simulink model "tdpSingleRobot"  (R2026b)
settings: Solver=FixedStepDiscrete  StopTime=15-P.dt  FixedStep=P.dt
model workspace (MAT data in the model file):
  P.L = 9
  P.W = 6
  P.goalD = 0.6
  P.goalW = 2.6
  P.goalAreaL = 1
  P.goalAreaW = 3
  P.penMark = 1.5
  P.centreD = 1.5
  P.border = 1
  P.penAreaL = 2
  P.penAreaW = 5
  P.ballR = 0.07
  P.ballDecel = 0.4
  P.ballRestit = 0.5
  P.ballRobotE = 0.3
  P.robotR = 0.15
  P.vFwd = 0.25
  P.vBack = 0.12
  P.vSide = 0.15
  P.wMax = 0.785398163397
  P.Kp = 0.8
  P.Kw = 2
  P.avoidR = 0.7
  P.avoidGain = 0.6
  P.ballAvoidR = 0.35
  P.approachDist = 0.45
  P.kickRange = 0.28
  P.stepInSpeed = 0.1
  P.kickAlign = 0.349065850399
  P.behindTol = 0.523598775598
  P.kickNoise = 0.10471975512
  P.kickCooldown = 1
  P.shotSpeed = 1.8
  P.dribbleSpeed = 0.6
  P.maxKickSpeed = 2.2
  P.roleHyst = 0.4
  P.shootDist = 3
  P.defDist = 1.8
  P.nPerTeam = 4
  P.dt = 0.05
  P.Tmatch = 600
  P.restartPause = 2
  P.outPause = 1
  P.drawEvery = 4
  P.realtime = 0
  P.dirSign = [1 -1]
  P.seed = 1
  P.mode : TdpMode (value not decoded)
  P.rulesProfile : TdpRules (value not decoded)
  P.maxObservationAge = 0.5
  P.walkValidity = 0.1
  P.kickPreparation = 0.2
  P.kickTimeout = 1
  P.recoverTime = 0.5
  P.alignEnter = 0.35
  P.alignExit = 0.45
  P.searchTurnRate = 0.3
  P.fieldOfView = 6.28318530718
  P.observationDelay = 0
  P.observationNoise = 0
  P.fixedStriker = 0
  P.tapSpeed = 0.3
  P.freezeDuringPause = 0
  P.contactIterations = 256
  P.restartOpponentDistance = 0.75
  P.contactTolerance = 1e-10
  feedback0(1).requestId = 0
  feedback0(1).status : TdpStatus (value not decoded)
  feedback0(1).stamp = 0
  feedback0(2).requestId = 0
  feedback0(2).status : TdpStatus (value not decoded)
  feedback0(2).stamp = 0
  feedback0(3).requestId = 0
  feedback0(3).status : TdpStatus (value not decoded)
  feedback0(3).stamp = 0
  feedback0(4).requestId = 0
  feedback0(4).status : TdpStatus (value not decoded)
  feedback0(4).stamp = 0
  feedback0(5).requestId = 0
  feedback0(5).status : TdpStatus (value not decoded)
  feedback0(5).stamp = 0
  feedback0(6).requestId = 0
  feedback0(6).status : TdpStatus (value not decoded)
  feedback0(6).stamp = 0
  feedback0(7).requestId = 0
  feedback0(7).status : TdpStatus (value not decoded)
  feedback0(7).stamp = 0
  feedback0(8).requestId = 0
  feedback0(8).status : TdpStatus (value not decoded)
  feedback0(8).stamp = 0
  singleIntent.type : TdpAction (value not decoded)
  singleIntent.target = [4.5 0]
  singleIntent.heading = 0
  singleIntent.speed = 1.8
  singleIntent.role : TdpRole (value not decoded)
  world0.robots(1).team = 1
  world0.robots(1).num = 1
  world0.robots(1).isGK = 1
  world0.robots(1).role : TdpRole (value not decoded)
  world0.robots(1).x = -1
  world0.robots(1).y = 0
  world0.robots(1).th = 0
  world0.robots(1).vxw = 0
  world0.robots(1).vyw = 0
  world0.robots(1).cool = 0
  world0.robots(2).team = 1
  world0.robots(2).num = 2
  world0.robots(2).isGK = 0
  world0.robots(2).role : TdpRole (value not decoded)
  world0.robots(2).x = 24
  world0.robots(2).y = 20
  world0.robots(2).th = 0
  world0.robots(2).vxw = 0
  world0.robots(2).vyw = 0
  world0.robots(2).cool = 0
  world0.robots(3).team = 1
  world0.robots(3).num = 3
  world0.robots(3).isGK = 0
  world0.robots(3).role : TdpRole (value not decoded)
  world0.robots(3).x = 26
  world0.robots(3).y = 20
  world0.robots(3).th = 0
  world0.robots(3).vxw = 0
  world0.robots(3).vyw = 0
  world0.robots(3).cool = 0
  world0.robots(4).team = 1
  world0.robots(4).num = 4
  world0.robots(4).isGK = 0
  world0.robots(4).role : TdpRole (value not decoded)
  world0.robots(4).x = 28
  world0.robots(4).y = 20
  world0.robots(4).th = 0
  world0.robots(4).vxw = 0
  world0.robots(4).vyw = 0
  world0.robots(4).cool = 0
  world0.robots(5).team = 2
  world0.robots(5).num = 1
  world0.robots(5).isGK = 1
  world0.robots(5).role : TdpRole (value not decoded)
  world0.robots(5).x = 30
  world0.robots(5).y = 20
  world0.robots(5).th = 3.14159265359
  world0.robots(5).vxw = 0
  world0.robots(5).vyw = 0
  world0.robots(5).cool = 0
  world0.robots(6).team = 2
  world0.robots(6).num = 2
  world0.robots(6).isGK = 0
  world0.robots(6).role : TdpRole (value not decoded)
  world0.robots(6).x = 32
  world0.robots(6).y = 20
  world0.robots(6).th = 3.14159265359
  world0.robots(6).vxw = 0
  world0.robots(6).vyw = 0
  world0.robots(6).cool = 0
  world0.robots(7).team = 2
  world0.robots(7).num = 3
  world0.robots(7).isGK = 0
  world0.robots(7).role : TdpRole (value not decoded)
  world0.robots(7).x = 34
  world0.robots(7).y = 20
  world0.robots(7).th = 3.14159265359
  world0.robots(7).vxw = 0
  world0.robots(7).vyw = 0
  world0.robots(7).cool = 0
  world0.robots(8).team = 2
  world0.robots(8).num = 4
  world0.robots(8).isGK = 0
  world0.robots(8).role : TdpRole (value not decoded)
  world0.robots(8).x = 36
  world0.robots(8).y = 20
  world0.robots(8).th = 3.14159265359
  world0.robots(8).vxw = 0
  world0.robots(8).vyw = 0
  world0.robots(8).cool = 0
  world0.ball.x = 0
  world0.ball.y = 0
  world0.ball.vx = 0
  world0.ball.vy = 0
  world0.referee.t = 0
  world0.referee.score = [0 0]
  world0.referee.lastTouch = 0
  world0.referee.pauseUntil = 0
  world0.referee.msg : TdpEvent (value not decoded)
  world0.referee.msgUntil = 2
  world0.referee.shots = [0 0]
  world0.referee.touchTime = [0 0]
  world0.actuator(1).seenId = 0
  world0.actuator(1).rejectedId = 0
  world0.actuator(1).active = 0
  world0.actuator(1).start = 0
  world0.actuator(1).target = [0 0]
  world0.actuator(1).speed = 0
  world0.actuator(1).feedback.requestId = 0
  world0.actuator(1).feedback.status : TdpStatus (value not decoded)
  world0.actuator(1).feedback.stamp = 0
  world0.actuator(1).executions = 0
  world0.actuator(2).seenId = 0
  world0.actuator(2).rejectedId = 0
  world0.actuator(2).active = 0
  world0.actuator(2).start = 0
  world0.actuator(2).target = [0 0]
  world0.actuator(2).speed = 0
  world0.actuator(2).feedback.requestId = 0
  world0.actuator(2).feedback.status : TdpStatus (value not decoded)
  world0.actuator(2).feedback.stamp = 0
  world0.actuator(2).executions = 0
  world0.actuator(3).seenId = 0
  world0.actuator(3).rejectedId = 0
  world0.actuator(3).active = 0
  world0.actuator(3).start = 0
  world0.actuator(3).target = [0 0]
  world0.actuator(3).speed = 0
  world0.actuator(3).feedback.requestId = 0
  world0.actuator(3).feedback.status : TdpStatus (value not decoded)
  world0.actuator(3).feedback.stamp = 0
  world0.actuator(3).executions = 0
  world0.actuator(4).seenId = 0
  world0.actuator(4).rejectedId = 0
  world0.actuator(4).active = 0
  world0.actuator(4).start = 0
  world0.actuator(4).target = [0 0]
  world0.actuator(4).speed = 0
  world0.actuator(4).feedback.requestId = 0
  world0.actuator(4).feedback.status : TdpStatus (value not decoded)
  world0.actuator(4).feedback.stamp = 0
  world0.actuator(4).executions = 0
  world0.actuator(5).seenId = 0
  world0.actuator(5).rejectedId = 0
  world0.actuator(5).active = 0
  world0.actuator(5).start = 0
  world0.actuator(5).target = [0 0]
  world0.actuator(5).speed = 0
  world0.actuator(5).feedback.requestId = 0
  world0.actuator(5).feedback.status : TdpStatus (value not decoded)
  world0.actuator(5).feedback.stamp = 0
  world0.actuator(5).executions = 0
  world0.actuator(6).seenId = 0
  world0.actuator(6).rejectedId = 0
  world0.actuator(6).active = 0
  world0.actuator(6).start = 0
  world0.actuator(6).target = [0 0]
  world0.actuator(6).speed = 0
  world0.actuator(6).feedback.requestId = 0
  world0.actuator(6).feedback.status : TdpStatus (value not decoded)
  world0.actuator(6).feedback.stamp = 0
  world0.actuator(6).executions = 0
  world0.actuator(7).seenId = 0
  world0.actuator(7).rejectedId = 0
  world0.actuator(7).active = 0
  world0.actuator(7).start = 0
  world0.actuator(7).target = [0 0]
  world0.actuator(7).speed = 0
  world0.actuator(7).feedback.requestId = 0
  world0.actuator(7).feedback.status : TdpStatus (value not decoded)
  world0.actuator(7).feedback.stamp = 0
  world0.actuator(7).executions = 0
  world0.actuator(8).seenId = 0
  world0.actuator(8).rejectedId = 0
  world0.actuator(8).active = 0
  world0.actuator(8).start = 0
  world0.actuator(8).target = [0 0]
  world0.actuator(8).speed = 0
  world0.actuator(8).feedback.requestId = 0
  world0.actuator(8).feedback.status : TdpStatus (value not decoded)
  world0.actuator(8).feedback.stamp = 0
  world0.actuator(8).executions = 0
  world0.active = [1 0 0 0 0 0 0 0]
  world0.lastCommands = [0  0  0; 0  0  0; 0  0  0; 0  0  0; 0  0  0; 0  0  0; 0  0  0; 0  0  0]
  world0.lastKick = 0
  world0.kickCount = 0
libraries: ControllerCore x1
settings Model: DataDictionary=TdpTypes.sldd  Creator=fayne  LastModifiedBy=fayne
settings DataIOCC: SaveOutput=off  SignalLogging=off
settings DebuggingCC: AlgebraicLoopMsg=error

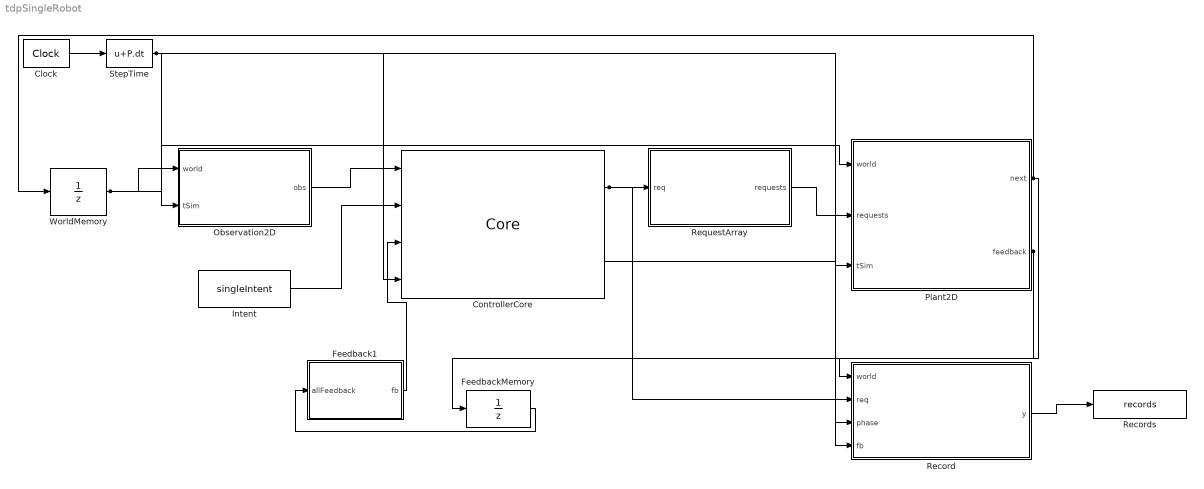
== system tdpSingleRobot ==
  Clock : DigitalClock  SampleTime=P.dt
  ControllerCore : ControllerCore/Core  SystemSampleTime=-1  VariantActivationTime=update diagram  EmptyChoice=off  PassThrough=off  PassThroughVariantControl=(default)  EmptyChoiceVariantControl=(default)  AllowFlexibleInterface=on  Latency=0  AutoFrameSizeCalculation=off
  Feedback1 : MATLAB Function  TreatAsAtomicUnit=on
  FeedbackMemory : UnitDelay  InitialCondition=feedback0  SampleTime=P.dt
  Intent : Constant  Value=singleIntent  OutDataTypeStr=Bus: IntentBus
  Observation2D : MATLAB Function  TreatAsAtomicUnit=on
  Plant2D : MATLAB Function  TreatAsAtomicUnit=on
  Record : MATLAB Function  TreatAsAtomicUnit=on
  Records : ToWorkspace  VariableName=records  SampleTime=-1
  RequestArray : MATLAB Function  TreatAsAtomicUnit=on
  StepTime : Bias  Bias=P.dt  SaturateOnIntegerOverflow=off
  WorldMemory : UnitDelay  InitialCondition=world0  SampleTime=P.dt
  wires:
  Clock/1 -> StepTime/1
  WorldMemory/1 -> Observation2D/1(world), Plant2D/1(world)
  StepTime/1 -> Observation2D/2(tSim), ControllerCore/4, Plant2D/3(tSim)
  Observation2D/1(obs) -> ControllerCore/1
  Intent/1 -> ControllerCore/2
  FeedbackMemory/1 -> Feedback1/1(allFeedback)
  Feedback1/1(fb) -> ControllerCore/3
  ControllerCore/1 -> RequestArray/1(req), Record/2(req)
  RequestArray/1(requests) -> Plant2D/2(requests)
  Plant2D/1(next) -> WorldMemory/1, Record/1(world)
  Plant2D/2(feedback) -> FeedbackMemory/1, Record/4(fb)
  ControllerCore/2 -> Record/3(phase)
  Record/1(y) -> Records/1

== matlab function tdpSingleRobot/Feedback1 ==
  data: allFeedback input Bus: FeedbackBus size=[1 8]; fb output Bus: FeedbackBus
function fb=f(allFeedback)
fb=allFeedback(1);
end

== matlab function tdpSingleRobot/Observation2D ==
  data: world input Bus: WorldBus; obs output Bus: ObservationBus; tSim input; P parameter
function obs=f(world,tSim,P)
obs=Observation2D(world,1,tSim,P);
end

== matlab function tdpSingleRobot/RequestArray ==
  data: req input Bus: RequestBus; requests output Bus: RequestBus size=[1 8]
function requests=f(req)
requests=repmat(req,1,8);
for i=2:8,requests(i).kind=TdpAction.Stop;requests(i).velocity=[0 0 0];end
end

== matlab function tdpSingleRobot/Plant2D ==
  data: world input Bus: WorldBus; next output Bus: WorldBus; requests input Bus: RequestBus size=[1 8]; tSim input; feedback output Bus: FeedbackBus size=[1 8]; P parameter
function [next,feedback]=f(world,requests,tSim,P)
[next,feedback]=Plant2D(world,requests,tSim,P);
end

== matlab function tdpSingleRobot/Record ==
  data: world input Bus: WorldBus; y output; req input Bus: RequestBus; phase input Enum: TdpPhase; fb input Bus: FeedbackBus
function y=f(world,req,phase,fb)
r=world.robots(1);b=world.ball;
y=[r.x r.y r.th b.x b.y b.vx b.vy double(world.kickCount) double(req.kind) double(req.requestId) double(phase) double(fb(1).status) double(fb(1).requestId) double(world.actuator(1).executions)];
end
